simulink model "PDW_TestBench_SIL"  (R2022b)
settings: Solver=FixedStepDiscrete  StartTime=0.0  StopTime=2  FixedStep=0.02  RelTol=1e-3
settings Model: Creator=chaym  LastModifiedBy=chaym

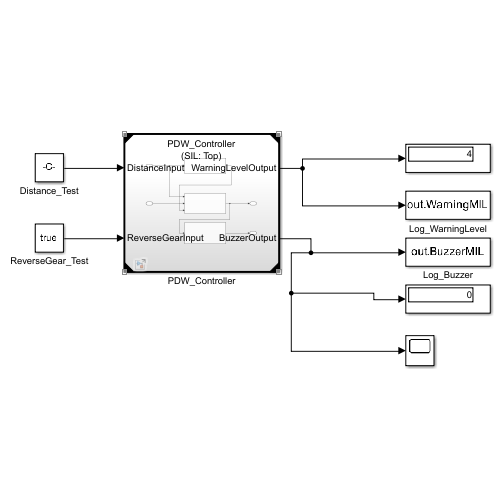
[thumbnail: Simulink's stored preview of the top-level diagram]
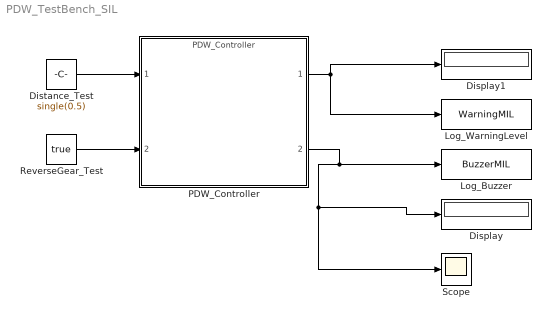
== system PDW_TestBench_SIL ==
  Display : Display
  Display1 : Display
  Distance_Test : Constant  Value=single(0.5)
  Log_Buzzer : ToWorkspace  VariableName=BuzzerMIL  SaveFormat=Timeseries  SampleTime=-1
  Log_WarningLevel : ToWorkspace  VariableName=WarningMIL  SaveFormat=Timeseries  SampleTime=-1
  PDW_Controller : ModelReference  ModelNameDialog=PDW_Controller  SimulationMode=Software-in-the-loop (SIL)  CodeInterface=Top model  ModelReferenceVersion=1.32
  ReverseGear_Test : Constant  Value=true  OutDataTypeStr=boolean
  Scope : Scope
  wires:
  Distance_Test/1 -> PDW_Controller/1
  ReverseGear_Test/1 -> PDW_Controller/2
  PDW_Controller/2 -> Display/1, Scope/1, Log_Buzzer/1
  PDW_Controller/1 -> Display1/1, Log_WarningLevel/1
